simulink model "send_receive"  (R2025a)
settings: Solver=FixedStepDiscrete  StartTime=0.0  StopTime=inf  RelTol=1e-3
model workspace (MAT data in the model file):
  board_ID = 1
undefined symbols (not defined in the file): canChannel
libraries: canmsglib x10, canlib x3
settings Model: Creator=sgirardi  LastModifiedBy=mfussi
settings DebuggingCC: UnconnectedInputMsg=warning  UnconnectedOutputMsg=warning  UnconnectedLineMsg=warning
settings ModelReferenceCC: EnableRefExpFcnMdlSchedulingChecks=on
settings RTWCC: GPUComputeCapability=3.5  DLArmComputeVersion=19.05

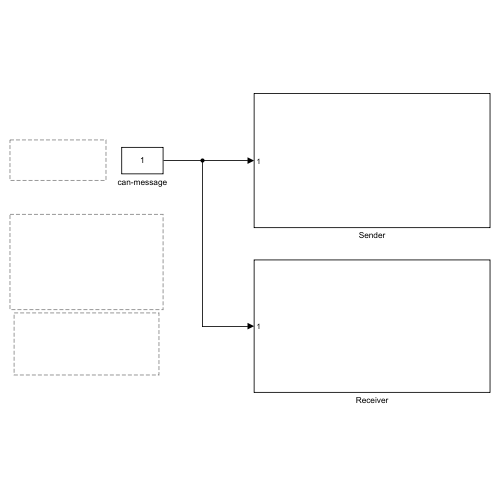
[thumbnail: Simulink's stored preview of the top-level diagram]
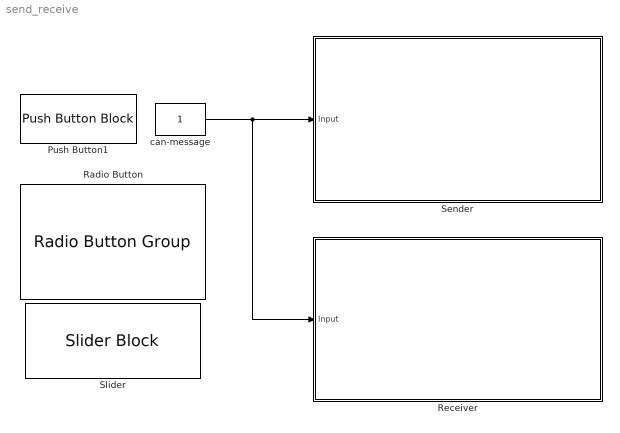
== system send_receive ==
  Push Button1 : PushButtonBlock  ButtonText=Send Messange  Icon=TurnSignalRight  IconAlignment=Right  IconOnColor=[0.0, 0.39215686274509803, 0.0]  IconOffColor=[0.0, 1.0, 0.0]  OffValue=0.000000
  Radio Button : RadioButtonGroup  SelectedLabel=set-control-mode-idle  ButtonGroupName=CAN Messages
  Receiver : Subsystem
  Sender : Subsystem
  Slider : SliderBlock  ScaleMin=-250  ScaleMax=250  TickInterval=100
  can-message : Constant
  wires:
  can-message/1 -> Receiver/1(Input), Sender/1(Input)

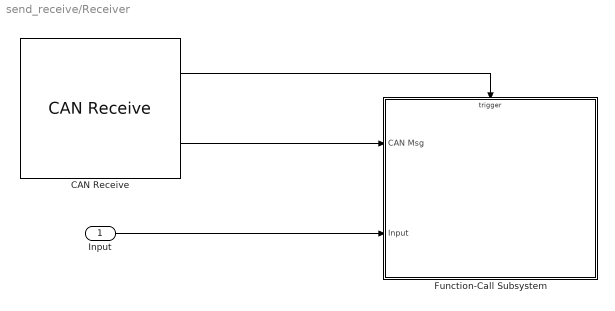
== system send_receive/Receiver ==
  Input : Inport
  CAN Receive : canlib/CAN Receive  BlockHandle=241410.0004  Device=MathWorks Virtual 1 (Channel 1)  DeviceMenu=MathWorks Virtual 1 (Channel 1)  ObjConstructor=canChannel('MathWorks', 'Virtual 1', 1)  EnableStandardIDsFilter=off  StdIDsCombo=Allow all  StandardIDs=0  EnableExtendedIDsFilter=off  ExtIDsCombo=Allow all  ExtendedIDs=0  SampleTime=0.01  MsgsPerTimestep=all  InternalFilterUpdateStatus=on  BusOutput=on
  Function-Call Subsystem : Subsystem  TreatAsAtomicUnit=on
  wires:
  CAN Receive/1 -> Function-Call Subsystem/Trigger
  CAN Receive/2 -> Function-Call Subsystem/1(CAN Msg)
  Input/1 -> Function-Call Subsystem/2(Input)

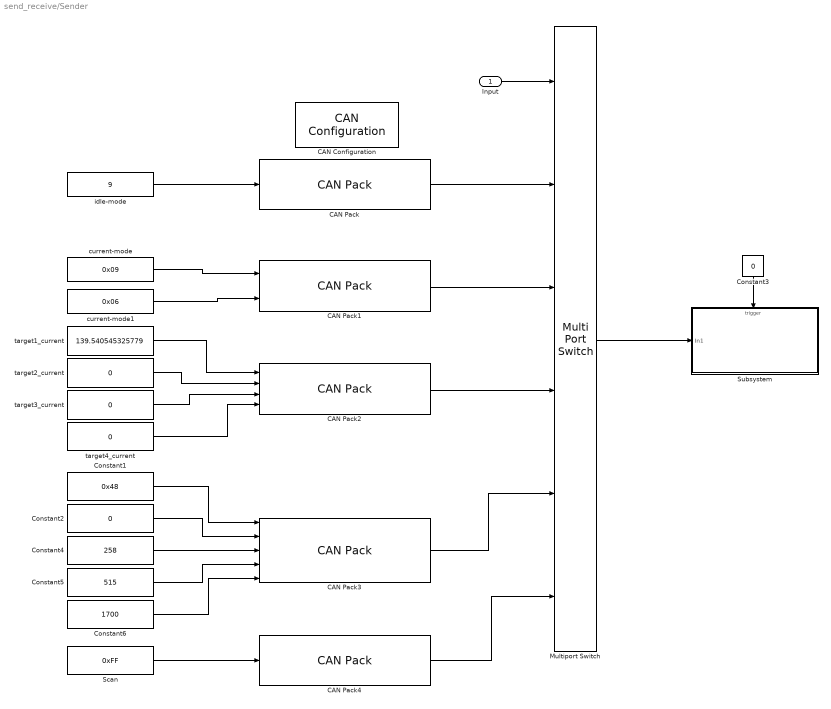
== system send_receive/Sender ==
  Input : Inport
  CAN Configuration : canlib/CAN Configuration  BlockHandle=241534.0004  Device=MathWorks Virtual 1 (Channel 1)  DeviceMenu=MathWorks Virtual 1 (Channel 1)  ObjConstructor=canChannel('MathWorks', 'Virtual 1', 1)  BusSpeed=500000  EnableBitParameters=off  AckMode=Normal
  CAN Pack : canmsglib/CAN Pack  MsgList=(none)  MsgName=CAN Idle  MsgIDType=Standard (11-bit identifier)  MsgIdentifier=board_ID  CANIDInput=off  MsgLength=2  Remote=off  ApplyMinMax=off  BusOutput=on  SignalInfo={ 'Idle', '0', '16', 'LE', 'unsigned', 'Standard', '0', '1', '0', '-Inf', 'Inf' }
      settings: DataFormat=manually specified signals
  CAN Pack1 : canmsglib/CAN Pack  MsgList=(none)  MsgName=CAN Current Mode  MsgIDType=Standard (11-bit identifier)  MsgIdentifier=board_ID  CANIDInput=off  MsgLength=2  Remote=off  ApplyMinMax=off  BusOutput=on  SignalInfo={ 'CMD', '0', '8', 'LE', 'unsigned', 'Standard', '0', '1', '0', '-Inf', 'Inf'; 'CTRL', '8', '8', 'LE', 'signed', 'Standard', '0', '1', '0', '-Inf', 'Inf' }
      settings: DataFormat=manually specified signals
  CAN Pack2 : canmsglib/CAN Pack  MsgList=(none)  MsgName=CAN Target  MsgIDType=Standard (11-bit identifier)  MsgIdentifier=0x10F  CANIDInput=off  MsgLength=8  Remote=off  ApplyMinMax=off  BusOutput=on  SignalInfo={ 'Target 1', '0', '16', 'LE', 'signed', 'Standard', '0', '1', '0', '-Inf', 'Inf'; 'Target 2', '16', '16', 'LE', 'signed', 'Standard', '0', '1', '0', '-Inf', 'Inf'; 'Target 3', '32', '16', 'LE', 'signed', 'Standard', '0', '1', '0', '-Inf', 'Inf'; 'Target 4', '48', '16', 'LE', 'signed', 'Standard', '0', '1', '0', '-Inf', 'Inf' }
      settings: DataFormat=manually specified signals
  CAN Pack3 : canmsglib/CAN Pack  MsgList=(none)  MsgName=CAN Limits  MsgIDType=Standard (11-bit identifier)  MsgIdentifier=board_ID  CANIDInput=off  MsgLength=8  Remote=off  ApplyMinMax=off  BusOutput=on  SignalInfo={ 'CMD', '0', '8', 'LE', 'unsigned', 'Standard', '0', '1', '0', '-Inf', 'Inf'; 'X', '8', '8', 'LE', 'unsigned', 'Standard', '0', '1', '0', '-Inf', 'Inf'; 'NOMINAL', '16', '16', 'LE', 'unsigned', 'Standard', '0', '1', '0', '-Inf', 'Inf'; 'PEAK', '32', '16', 'LE', 'unsigned', 'Standard', '0', '1', '0', '-Inf', 'Inf'; 'OVERLOAD', '48', '16', 'LE', 'unsigned', 'Standard', '0', '1', '0', '-Inf', 'Inf' }
      settings: DataFormat=manually specified signals
  CAN Pack4 : canmsglib/CAN Pack  MsgList=(none)  MsgName=CAN Msg  MsgIDType=Standard (11-bit identifier)  MsgIdentifier=0x70F  CANIDInput=off  MsgLength=1  Remote=off  ApplyMinMax=off  BusOutput=on  SignalInfo={}
      settings: DataFormat=raw data
  Constant1 : Constant  Value=0x48  OutDataTypeStr=Inherit: Inherit via back propagation
  Constant2 : Constant  Value=0  OutDataTypeStr=Inherit: Inherit via back propagation
  Constant3 : Constant  Value=0
  Constant4 : Constant  Value=258  OutDataTypeStr=Inherit: Inherit via back propagation
  Constant5 : Constant  Value=515  OutDataTypeStr=Inherit: Inherit via back propagation
  Constant6 : Constant  Value=1700  OutDataTypeStr=Inherit: Inherit via back propagation
  Multiport Switch : MultiPortSwitch  Inputs=5  SaturateOnIntegerOverflow=off  InputSameDT=off
  Scan : Constant  Value=0xFF
  Subsystem : Subsystem
  current-mode : Constant  Value=0x09  OutDataTypeStr=Inherit: Inherit via back propagation
  current-mode1 : Constant  Value=0x06  OutDataTypeStr=Inherit: Inherit via back propagation
  idle-mode : Constant  Value=9  OutDataTypeStr=Inherit: Inherit via back propagation
  target1_current : Constant  Value=139.540545325779  OutDataTypeStr=Inherit: Inherit via back propagation
  target2_current : Constant  Value=0  OutDataTypeStr=Inherit: Inherit via back propagation
  target3_current : Constant  Value=0  OutDataTypeStr=Inherit: Inherit via back propagation
  target4_current : Constant  Value=0  OutDataTypeStr=Inherit: Inherit via back propagation
  wires:
  CAN Pack/1 -> Multiport Switch/2
  CAN Pack1/1 -> Multiport Switch/3
  CAN Pack2/1 -> Multiport Switch/4
  Input/1 -> Multiport Switch/1
  idle-mode/1 -> CAN Pack/1
  current-mode/1 -> CAN Pack1/1
  target1_current/1 -> CAN Pack2/1
  Constant1/1 -> CAN Pack3/1
  CAN Pack3/1 -> Multiport Switch/5
  Scan/1 -> CAN Pack4/1
  CAN Pack4/1 -> Multiport Switch/6
  Constant3/1 -> Subsystem/Trigger
  Multiport Switch/1 -> Subsystem/1(In1)
  Constant2/1 -> CAN Pack3/2
  Constant4/1 -> CAN Pack3/3
  Constant5/1 -> CAN Pack3/4
  Constant6/1 -> CAN Pack3/5
  current-mode1/1 -> CAN Pack1/2
  target2_current/1 -> CAN Pack2/2
  target3_current/1 -> CAN Pack2/3
  target4_current/1 -> CAN Pack2/4

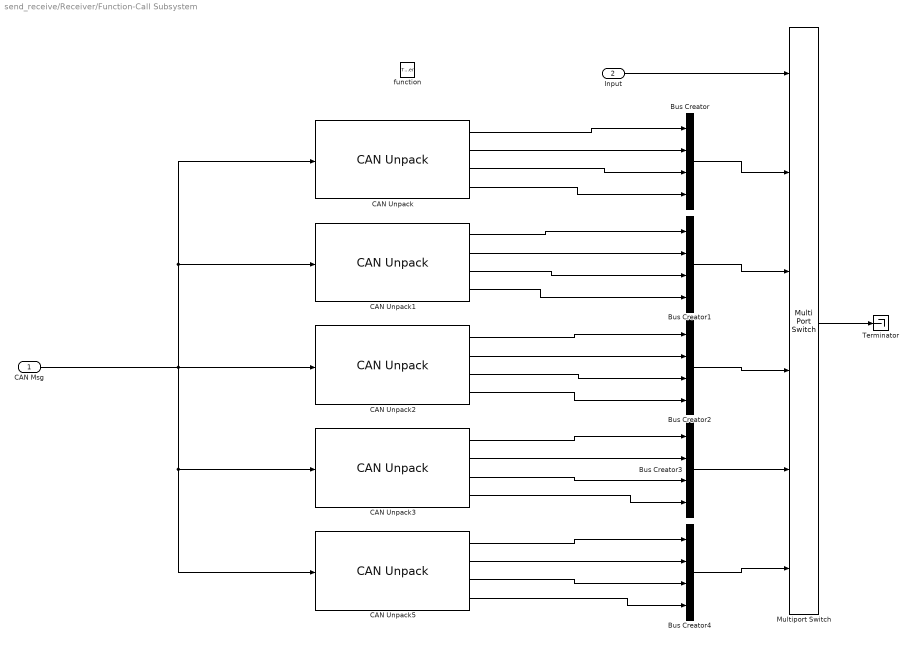
== system send_receive/Receiver/Function-Call Subsystem ==
  CAN Msg : Inport
  Input : Inport  Port=2
  function : TriggerPort  TriggerType=function-call  VariantControl=(inherit)
  Bus Creator{,1..4} (5 alike) : BusCreator  Inputs=4
  CAN Unpack : canmsglib/CAN Unpack  MsgList=(none)  MsgName=CAN Idle  MsgIDType=Standard (11-bit identifier)  MsgIdentifier=0x710  MsgLength=5  SignalInfo={}  IDPort=on  TimestampPort=on  ErrorPort=off  RemotePort=off  LengthPort=on  StatusPort=off  ApplyMinMax=off
      settings: DataFormat=raw data
  CAN Unpack1 : canmsglib/CAN Unpack  MsgList=(none)  MsgName=CAN Current Mode  MsgIDType=Standard (11-bit identifier)  MsgIdentifier=1824  MsgLength=5  SignalInfo={}  IDPort=on  TimestampPort=on  ErrorPort=off  RemotePort=off  LengthPort=on  StatusPort=off  ApplyMinMax=off
      settings: DataFormat=raw data
  CAN Unpack2 : canmsglib/CAN Unpack  MsgList=(none)  MsgName=CAN Target  MsgIDType=Standard (11-bit identifier)  MsgIdentifier=1824  MsgLength=5  SignalInfo={}  IDPort=on  TimestampPort=on  ErrorPort=off  RemotePort=off  LengthPort=on  StatusPort=off  ApplyMinMax=off
      settings: DataFormat=raw data
  CAN Unpack3 : canmsglib/CAN Unpack  MsgList=(none)  MsgName=CAN Limits  MsgIDType=Standard (11-bit identifier)  MsgIdentifier=1824  MsgLength=5  SignalInfo={}  IDPort=on  TimestampPort=on  ErrorPort=off  RemotePort=off  LengthPort=on  StatusPort=off  ApplyMinMax=off
      settings: DataFormat=raw data
  CAN Unpack5 : canmsglib/CAN Unpack  MsgList=(none)  MsgName=CAN Scan  MsgIDType=Standard (11-bit identifier)  MsgIdentifier=0x710  MsgLength=5  SignalInfo={}  IDPort=on  TimestampPort=on  ErrorPort=off  RemotePort=off  LengthPort=on  StatusPort=off  ApplyMinMax=off
      settings: DataFormat=raw data
  Multiport Switch : MultiPortSwitch  Inputs=5  SaturateOnIntegerOverflow=off  InputSameDT=off
  Terminator : Terminator
  wires:
  CAN Msg/1 -> CAN Unpack5/1, CAN Unpack3/1, CAN Unpack2/1, CAN Unpack1/1, CAN Unpack/1
  Multiport Switch/1 -> Terminator/1
  CAN Unpack/3 -> Bus Creator/3
  CAN Unpack/4 -> Bus Creator/4
  CAN Unpack/2 -> Bus Creator/2
  CAN Unpack1/1 -> Bus Creator1/1
  CAN Unpack1/4 -> Bus Creator1/4
  CAN Unpack1/3 -> Bus Creator1/3
  CAN Unpack1/2 -> Bus Creator1/2
  CAN Unpack2/1 -> Bus Creator2/1
  CAN Unpack2/4 -> Bus Creator2/4
  CAN Unpack2/3 -> Bus Creator2/3
  CAN Unpack2/2 -> Bus Creator2/2
  CAN Unpack3/4 -> Bus Creator3/4
  CAN Unpack3/3 -> Bus Creator3/3
  CAN Unpack3/2 -> Bus Creator3/2
  CAN Unpack5/4 -> Bus Creator4/4
  CAN Unpack5/3 -> Bus Creator4/3
  CAN Unpack5/2 -> Bus Creator4/2
  Input/1 -> Multiport Switch/1
  CAN Unpack/1 -> Bus Creator/1
  Bus Creator/1 -> Multiport Switch/2
  Bus Creator1/1 -> Multiport Switch/3
  Bus Creator2/1 -> Multiport Switch/4
  CAN Unpack3/1 -> Bus Creator3/1
  CAN Unpack5/1 -> Bus Creator4/1
  Bus Creator4/1 -> Multiport Switch/6
  Bus Creator3/1 -> Multiport Switch/5

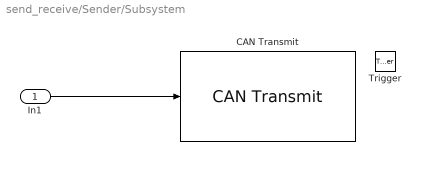
== system send_receive/Sender/Subsystem ==
  In1 : Inport
  Trigger : TriggerPort  VariantControl=(inherit)  PortDimensions=1
  CAN Transmit : canlib/CAN Transmit  BlockHandle=241586.0004  Device=MathWorks Virtual 1 (Channel 1)  DeviceMenu=MathWorks Virtual 1 (Channel 1)  ObjConstructor=canChannel('MathWorks', 'Virtual 1', 1)  EnableEventTransmit=off  EnablePeriodicTransmit=off  MessagePeriod=1.000
  wires:
  In1/1 -> CAN Transmit/1
